simulink model "fi_afc"  (R2026a)
settings: Solver=ode15s  StopTime=simTime  FixedStep=5e-05  RelTol=1e-06  AbsTol=1e-06
undefined symbols (not defined in the file or in its folder): AF_sensor_tol, fault_time, fuel_inj_tol, MAF_sensor_tol, measureTime, simTime, spec_num
Description:
  | Modeling Engine Timing Using Triggered Subsystems
  | 
  | This example presents a model of a four-cylinder spark ignition engine
  | and demonstrates Simulink(R) capabilities to model an internal combustion
  | engine from the throttle to the crankshaft output. We used well-defined
  | physical principles supplemented, where appropriate, with empirical
  | relationships that describe the systems dynamic behavior without
  | introducing unnecessary complexity.
settings Model: ExtModeTrigMode=oneshot  ExtModeArmWhenConnect=off  ExtModeAutoUpdateStatusClock=off  Creator=The MathWorks Inc.  LastModifiedBy=harry_31916
settings SolverCC: ConsecutiveZCsStepRelTol=2.8421709430404e-13
settings DataIOCC: ExternalInput=[t__,u__]  InitialState=[]  LoadExternalInput=on  SaveFormat=StructureWithTime  SignalLoggingSaveFormat=ModelDataLogs  StateSaveName=x  SignalLoggingName=sldemo_engine_output
settings OptimizationCC: BooleanDataType=off  InitFltsAndDblsToZero=on  BufferReusableBoundary=off
settings DebuggingCC: SignalInfNanChecking=warning  SaveWithParameterizedLinksMsg=none  UnderspecifiedInitializationDetection=Classic  SignalResolutionControl=TryResolveAllWithWarning  InheritedTsInSrcMsg=none  MultiTaskDSMMsg=warning  MultiTaskCondExecSysMsg=none  SigSpecEnsureSampleTimeMsg=none  IntegerOverflowMsg=none  ParameterPrecisionLossMsg=none  UniqueDataStoreMsg=warning  IntegerSaturationMsg=none
settings HardwareCC: ProdHWDeviceType=32-bit Generic
settings GRTTargetCC: TargetFcnLib=ansi_tfl_tmw.mat  CombineOutputUpdateFcns=off  GRTInterface=on
settings ConfigComp: CovMetricSettings=d

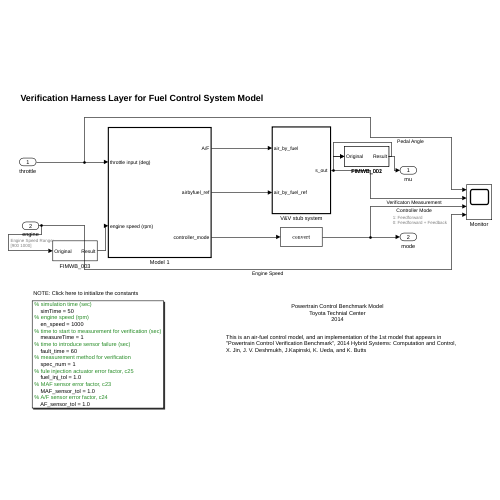
[thumbnail: Simulink's stored preview of the top-level diagram]
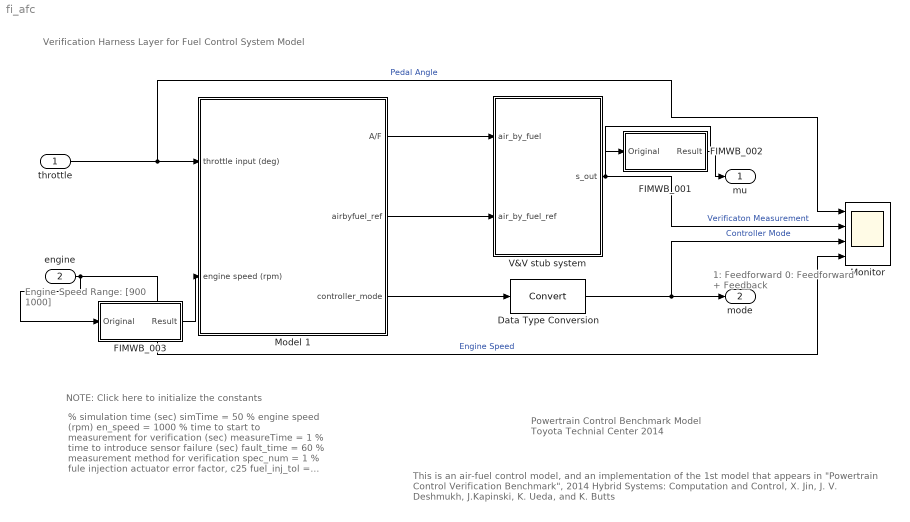
== system fi_afc ==
  note: 1: Feedforward
      | 0: Feedforward + Feedback
  note: NOTE: Click here to initialize the constants
  note: This is an air-fuel control model, and an implementation of the 1st model that appears in
      | "Powertrain Control Verification Benchmark", 2014 Hybrid Systems: Computation and Control,
      | X. Jin, J. V. Deshmukh, J.Kapinski, K. Ueda, and K. Butts
  note: % simulation time (sec)
      |     simTime = 50
      | % engine speed (rpm)
      |     en_speed = 1000
      | % time to start to measurement for verification (sec)
      |     measureTime = 1
      | % time to introduce sensor failure (sec)
      |     fault_time = 60
      | % measurement method for verification
      |     spec_num = 1
      | % fule injection actuator error factor, c25
      |     fuel_inj_tol = 1.0
      | % MAF sensor error factor, c23
      |     MAF_sensor_tol = 1.0
      | % A/F sensor error factor, c24
      |     AF_sensor_tol = 1.0
  note: Engine Speed Range:
      | [900 1000]
  note: Powertrain Control Benchmark Model
      | Toyota Technial Center
      | 2014
  note: Verification Harness Layer for Fuel Control System Model
  throttle : Inport  Interpolate=off
  engine : Inport  Port=2  Interpolate=off
  Data Type Conversion : DataTypeConversion  SaturateOnIntegerOverflow=off  RndMeth=Floor
  FIMWB_001 : Subsystem  Tag=fimwb.fault.1
  FIMWB_002 : Subsystem  Tag=fimwb.fault.2
  FIMWB_003 : Subsystem  Tag=fimwb.fault.3
  Model 1 : Subsystem  Priority=1  TreatAsAtomicUnit=on
  "Monitor " : Scope  NumInputPorts=4
      settings: TimeSpan=50  ActiveDisplayYMinimum=0  ActiveDisplayYMaximum=55
  V&V stub system : Subsystem  TreatAsAtomicUnit=on
  mu : Outport  VectorParamsAs1DForOutWhenUnconnected=off
  mode : Outport  Port=2  VectorParamsAs1DForOutWhenUnconnected=off
  wires:
  V&V stub system/1("s_out ") -> "Monitor "/2, FIMWB_001/1(Original)  "Verificaton Measurement"
  Model 1/1(A/F) -> V&V stub system/1("air_by_fuel ")
  engine/1 -> "Monitor "/4, FIMWB_003/1(Original)  "Engine Speed"
  throttle/1 -> "Monitor "/1, Model 1/1(throttle input (deg))  "Pedal Angle"
  Model 1/3(controller_mode) -> Data Type Conversion/1
  Data Type Conversion/1 -> "Monitor "/3, mode/1  "Controller Mode"
  Model 1/2(airbyfuel_ref) -> V&V stub system/2(air_by_fuel_ref)
  FIMWB_001/1(Result) -> FIMWB_002/1(Original)
  FIMWB_002/1(Result) -> mu/1
  FIMWB_003/1(Result) -> Model 1/2(engine speed (rpm))

== system fi_afc/FIMWB_001 ==
  Original : Inport
  Bias : Bias  Bias=-0.125  SaturateOnIntegerOverflow=off
  OutputType : DataTypeConversion  OutDataTypeStr=double  RndMeth=Round
  Result : Outport
  wires:
  Original/1 -> Bias/1
  Bias/1 -> OutputType/1
  OutputType/1 -> Result/1

== system fi_afc/FIMWB_002 ==
  Original : Inport
  Gain : Gain  Gain=1.5  OutDataTypeStr=Inherit: Same as input
  OutputType : DataTypeConversion  OutDataTypeStr=double  RndMeth=Round
  Result : Outport
  wires:
  Original/1 -> Gain/1
  Gain/1 -> OutputType/1
  OutputType/1 -> Result/1

== system fi_afc/FIMWB_003 ==
  Original : Inport
  Bias : Bias  Bias=0.015625  SaturateOnIntegerOverflow=off
  OutputType : DataTypeConversion  OutDataTypeStr=double  RndMeth=Round
  Result : Outport
  wires:
  Original/1 -> Bias/1
  Bias/1 -> OutputType/1
  OutputType/1 -> Result/1

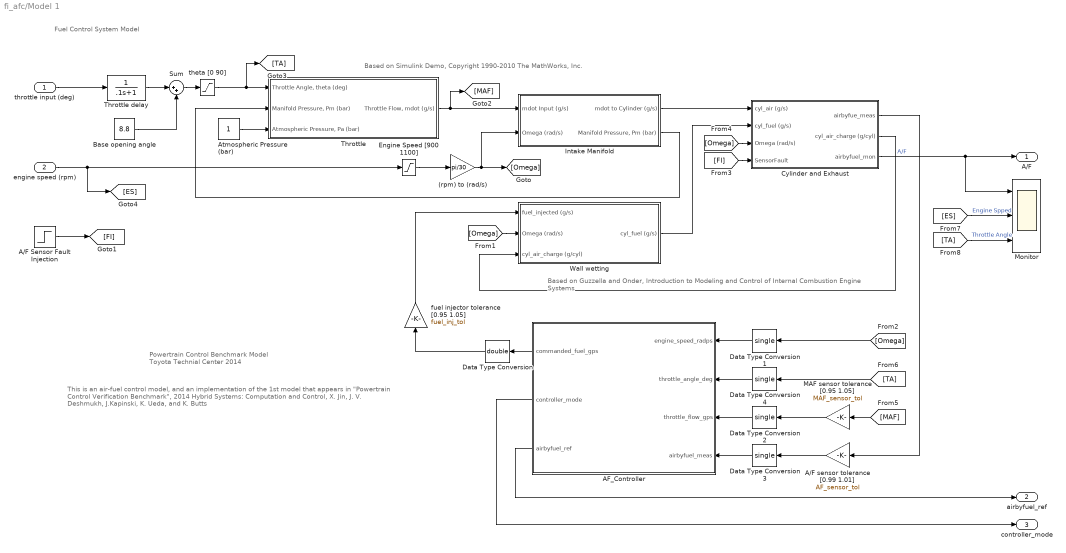
== system fi_afc/Model 1 ==
  note: Based on Simulink Demo, Copyright 1990-2010 The MathWorks, Inc.
  note: Based on Guzzella and Onder, Introduction to Modeling and Control of Internal Combustion Engine Systems
  note: Fuel Control System Model
  note: This is an air-fuel control model, and an implementation of the 1st model that appears in
      | "Powertrain Control Verification Benchmark", 2014 Hybrid Systems: Computation and Control,
      | X. Jin, J. V. Deshmukh, J.Kapinski, K. Ueda, and K. Butts
  note: Powertrain Control Benchmark Model
      | Toyota Technial Center
      | 2014
  throttle input (deg) : Inport  Description=[0, 81.2]
      settings: AttributesFormatString=%<Description>
  engine speed (rpm) : Inport  Description=[900,1100]  Port=2
      settings: AttributesFormatString=%<Description>
  (rpm) to (rad/s) : Gain  Gain=pi/30
  A/F Sensor Fault Injection : Step  Time=fault_time  SampleTime=0
      settings: AttributesFormatString=1: Failure\n0: Normal
  A/F sensor tolerance [0.99 1.01] : Gain  Gain=AF_sensor_tol
  AF_Controller : Subsystem  TreatAsAtomicUnit=on
  Atmospheric Pressure (bar) : Constant
  Base opening angle : Constant  Value=8.8
  Cylinder and Exhaust : Subsystem
  Data Type Conversion : DataTypeConversion  OutDataTypeStr=double  SaturateOnIntegerOverflow=off  RndMeth=Floor
  Data Type Conversion{1..4} (4 alike) : DataTypeConversion  OutDataTypeStr=single  SaturateOnIntegerOverflow=off  RndMeth=Floor
  Engine Speed [900 1100] : Saturate  UpperLimit=1100  LowerLimit=900
  Intake Manifold : Subsystem
  MAF sensor tolerance [0.95 1.05] : Gain  Gain=MAF_sensor_tol
  Monitor : Scope  NumInputPorts=3
      settings: TimeSpan=85  ActiveDisplayYMinimum=11.75  ActiveDisplayYMaximum=14.75
  Sum : Sum  Inputs=|++
  Throttle : Subsystem
  Throttle delay : TransferFcn  Denominator=[.1 1]
  Wall wetting : Subsystem
  fuel injector tolerance [0.95 1.05] : Gain  Gain=fuel_inj_tol
  theta [0 90] : Saturate  UpperLimit=90  LowerLimit=0
  A/F : Outport  VectorParamsAs1DForOutWhenUnconnected=off
  airbyfuel_ref : Outport  Port=2  VectorParamsAs1DForOutWhenUnconnected=off
  controller_mode : Outport  Port=3  VectorParamsAs1DForOutWhenUnconnected=off
  wires:
  (rpm) to (rad/s)/1 -> [Omega], Intake Manifold/2(Omega (rad/s))
  Data Type Conversion/1 -> fuel injector tolerance [0.95 1.05]/1
  theta [0 90]/1 -> Throttle/1("Throttle Angle, theta (deg)"), [TA]
  Engine Speed [900 1100]/1 -> (rpm) to (rad/s)/1
  Cylinder and Exhaust/3("airbyfuel_mon ") -> A/F/1, Monitor/1  "A/F"
  Data Type Conversion2/1 -> AF_Controller/3(throttle_flow_gps)
  Data Type Conversion3/1 -> AF_Controller/4(airbyfuel_meas)
  A/F sensor tolerance [0.99 1.01]/1 -> Data Type Conversion3/1
  [MAF] -> MAF sensor tolerance [0.95 1.05]/1
  Cylinder and Exhaust/1(airbyfue_meas) -> A/F sensor tolerance [0.99 1.01]/1
  Throttle/1("Throttle Flow, mdot (g/s)") -> [MAF], Intake Manifold/1(mdot Input (g/s))
  Intake Manifold/2("Manifold Pressure, Pm (bar)") -> Throttle/2("Manifold Pressure, Pm (bar)")
  Atmospheric Pressure (bar)/1 -> Throttle/3("Atmospheric Pressure, Pa (bar) ")
  Wall wetting/1(cyl_fuel (g/s)) -> Cylinder and Exhaust/2(cyl_fuel (g/s))
  Intake Manifold/1(mdot to Cylinder (g/s)) -> Cylinder and Exhaust/1(cyl_air (g/s))
  [Omega] -> Cylinder and Exhaust/3(Omega (rad/s))
  [Omega] -> Wall wetting/2(Omega (rad/s))
  Cylinder and Exhaust/2(cyl_air_charge (g/cyl)) -> Wall wetting/3(cyl_air_charge (g/cyl))
  [Omega] -> Data Type Conversion1/1
  fuel injector tolerance [0.95 1.05]/1 -> Wall wetting/1(fuel_injected (g/s))
  MAF sensor tolerance [0.95 1.05]/1 -> Data Type Conversion2/1
  AF_Controller/1(commanded_fuel_gps) -> Data Type Conversion/1
  Data Type Conversion1/1 -> AF_Controller/1(engine_speed_radps)
  A/F Sensor Fault Injection/1 -> [FI]
  [FI] -> Cylinder and Exhaust/4(SensorFault)
  [TA] -> Data Type Conversion4/1
  Data Type Conversion4/1 -> AF_Controller/2(throttle_angle_deg)
  throttle input (deg)/1 -> Throttle delay/1
  engine speed (rpm)/1 -> [ES], Engine Speed [900 1100]/1
  [TA] -> Monitor/3  "Throttle Angle"
  Throttle delay/1 -> Sum/1
  Base opening angle/1 -> Sum/2
  Sum/1 -> theta [0 90]/1
  AF_Controller/2(controller_mode) -> controller_mode/1
  AF_Controller/3(airbyfuel_ref) -> airbyfuel_ref/1
  [ES] -> Monitor/2  "Engine Spped"

== system fi_afc/V&V stub system ==
  "air_by_fuel " : Inport  OutDataTypeStr=double
  air_by_fuel_ref : Inport  Port=2
  Calcuate Error : Subsystem  Priority=20  TreatAsAtomicUnit=on
  Constant : Constant  Value=0.5
  Data Type Conversion : DataTypeConversion  OutDataTypeStr=double  SaturateOnIntegerOverflow=off  RndMeth=Floor
  MeasureOn : Step  Time=measureTime  SampleTime=0
  Relational Operator : RelationalOperator  Operator=>  OutDataTypeStr=boolean  InputSameDT=off
  spec_num : Constant  Value=spec_num  OutDataTypeStr=uint8
  "s_out " : Outport  VectorParamsAs1DForOutWhenUnconnected=off
  wires:
  Calcuate Error/1("s_out ") -> "s_out "/1
  MeasureOn/1 -> Relational Operator/1
  Constant/1 -> Relational Operator/2
  Relational Operator/1 -> Calcuate Error/Enable
  spec_num/1 -> Calcuate Error/2(spec_num)
  "air_by_fuel "/1 -> Calcuate Error/1("air_by_fuel ")
  air_by_fuel_ref/1 -> Data Type Conversion/1
  Data Type Conversion/1 -> Calcuate Error/3(air_by_fuel_ref)

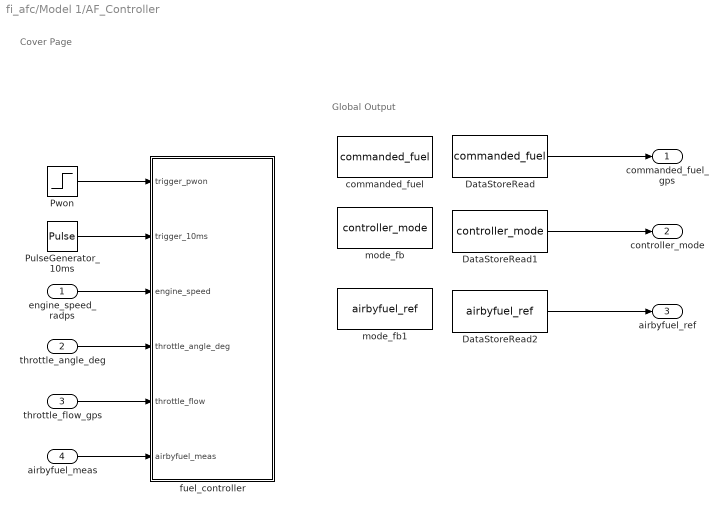
== system fi_afc/Model 1/AF_Controller ==
  note: Global Output
  note: Cover Page
  engine_speed_radps : Inport
  throttle_angle_deg : Inport  Port=2
  throttle_flow_gps : Inport  Port=3
  airbyfuel_meas : Inport  Port=4
  DataStoreRead : DataStoreRead  Priority=2  DataStoreName=commanded_fuel  IndexOptions=Index vector (dialog)  Indices=1  OutputSizes=1
  DataStoreRead1 : DataStoreRead  Priority=2  DataStoreName=controller_mode  IndexOptions=Index vector (dialog)  Indices=1  OutputSizes=1
  DataStoreRead2 : DataStoreRead  Priority=2  DataStoreName=airbyfuel_ref  IndexOptions=Index vector (dialog)  Indices=1  OutputSizes=1
  PulseGenerator_10ms : DiscretePulseGenerator  PulseType=Time based  Period=0.01  PulseWidth=50  PhaseDelay=0.01
  Pwon : Step  Time=0.001  SampleTime=0
  commanded_fuel : DataStoreMemory  DataStoreName=commanded_fuel  InitialValue=0.1726  ShowAdditionalParam=off  OutDataTypeStr=single
      settings: AttributesFormatString=commanded_fuel
  fuel_controller : Subsystem  Priority=1  TreatAsAtomicUnit=on
      settings: AttributesFormatString=Priority = %<Priority>
  mode_fb : DataStoreMemory  DataStoreName=controller_mode  ShowAdditionalParam=off  OutDataTypeStr=boolean
      settings: AttributesFormatString=controller_mode
  mode_fb1 : DataStoreMemory  DataStoreName=airbyfuel_ref  ShowAdditionalParam=off  OutDataTypeStr=single
  commanded_fuel_gps : Outport  VectorParamsAs1DForOutWhenUnconnected=off
  controller_mode : Outport  Port=2  VectorParamsAs1DForOutWhenUnconnected=off
  airbyfuel_ref : Outport  Port=3  VectorParamsAs1DForOutWhenUnconnected=off
  wires:
  DataStoreRead/1 -> commanded_fuel_gps/1
  airbyfuel_meas/1 -> fuel_controller/6(airbyfuel_meas)
  throttle_flow_gps/1 -> fuel_controller/5(throttle_flow)
  engine_speed_radps/1 -> fuel_controller/3(engine_speed)
  Pwon/1 -> fuel_controller/1(trigger_pwon)
  throttle_angle_deg/1 -> fuel_controller/4(throttle_angle_deg)
  PulseGenerator_10ms/1 -> fuel_controller/2(trigger_10ms)
  DataStoreRead1/1 -> controller_mode/1
  DataStoreRead2/1 -> airbyfuel_ref/1

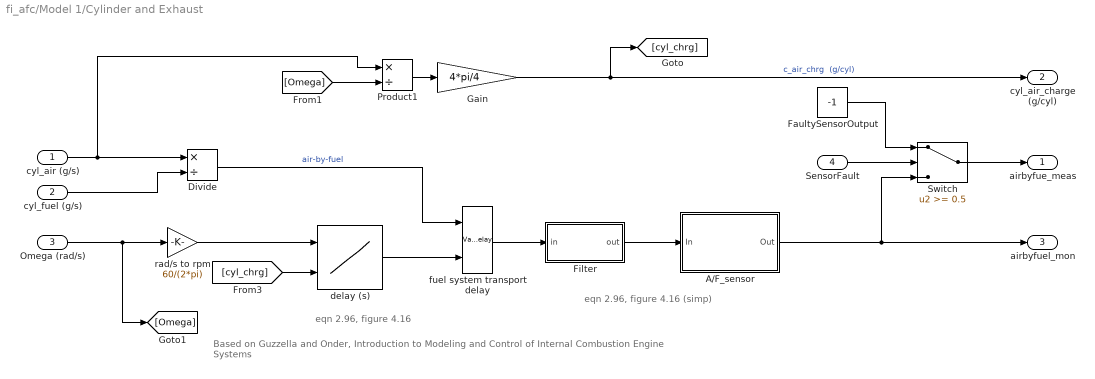
== system fi_afc/Model 1/Cylinder and Exhaust ==
  note: Based on Guzzella and Onder, Introduction to Modeling and Control of Internal Combustion Engine Systems
  note: eqn 2.96, figure 4.16
  note: eqn 2.96, figure 4.16 (simp)
  cyl_air (g/s) : Inport
  cyl_fuel (g/s) : Inport  Port=2
  Omega (rad/s) : Inport  Port=3
  SensorFault : Inport  Port=4
  A/F_sensor : Subsystem
  Divide : Product  Inputs=*/
  FaultySensorOutput : Constant  Value=-1
  Filter : Subsystem
  Gain : Gain  Gain=4*pi/4
  Product1 : Product  Inputs=*/  RndMeth=Zero
  Switch : Switch  Threshold=0.5  SaturateOnIntegerOverflow=off  InputSameDT=off
  delay (s) : Lookup_n-D  BreakpointsForDimension1=[800,1000,1500,2000,3000]  BreakpointsForDimension2=[0.05,0.15,0.2,0.25]  Table=reshape([0.8,0.6,0.4,0.3,0.2,0.4,0.3,0.2,0.2,0.2,0.3,0.25,0.2,0.2,0.2,0.25,0.2,0.2,0.2,0.2],5,4)  UseLastTableValue=on  RndMeth=Simplest
      settings: InputPortMap=u0,u1
  fuel system transport delay : VariableTransportDelay  VariableDelayType=Variable transport delay  MaximumDelay=10  InitialOutput=14.7  MaximumPoints=20480
  rad/s to rpm : Gain  Gain=60/(2*pi)
  airbyfue_meas : Outport  VectorParamsAs1DForOutWhenUnconnected=off
  cyl_air_charge (g/cyl) : Outport  Port=2  VectorParamsAs1DForOutWhenUnconnected=off
  "airbyfuel_mon " : Outport  Port=3  VectorParamsAs1DForOutWhenUnconnected=off
  wires:
  cyl_air (g/s)/1 -> Divide/1, Product1/1
  [Omega] -> Product1/2
  Product1/1 -> Gain/1
  Gain/1 -> [cyl_chrg], cyl_air_charge (g/cyl)/1  "c_air_chrg  (g/cyl)"
  [cyl_chrg] -> delay (s)/2
  cyl_fuel (g/s)/1 -> Divide/2
  Omega (rad/s)/1 -> [Omega], rad/s to rpm/1
  rad/s to rpm/1 -> delay (s)/1
  delay (s)/1 -> fuel system transport delay/2
  fuel system transport delay/1 -> Filter/1(in)
  Switch/1 -> airbyfue_meas/1
  Divide/1 -> fuel system transport delay/1  "air-by-fuel"
  Filter/1(out) -> A/F_sensor/1(In)
  FaultySensorOutput/1 -> Switch/1
  SensorFault/1 -> Switch/2
  A/F_sensor/1(Out) -> Switch/3, "airbyfuel_mon "/1

== system fi_afc/Model 1/Intake Manifold ==
  note: Intake Manifold Vacuum
  note: Based on Simulink Demo, Copyright 1990-2010 The MathWorks, Inc.
  mdot Input (g/s) : Inport
  Omega (rad/s) : Inport  Port=2
  Gain2 : Gain  Gain=0.9  ParamDataTypeStr=single  OutDataTypeStr=Inherit: Inherit via back propagation  RndMeth=Simplest  SaturateOnIntegerOverflow=on
      settings: AttributesFormatString=pumping tolerance [0.9 1.1]
  Mux : Mux  Inputs=2
  Pumping : Fcn  Expr=-0.366 + 0.08979*u[1]*u[2] - 0.0337*u[2]*u[1]*u[1] + 0.0001*u[1]*u[2]*u[2]
  RT/Vm : Gain  Gain=0.41328  SaturateOnIntegerOverflow=on  OutDataTypeStr=Inherit: Same as input  ParamDataTypeStr=Inherit: Same as input
  Sum : Sum  Inputs=|+-  InputSameDT=on  SaturateOnIntegerOverflow=on  OutDataTypeStr=Inherit: Same as first input
  p0 = 0.543 (bar) : Integrator  InitialCondition=0.982
  mdot to Cylinder (g/s) : Outport  InitialOutput=0  VectorParamsAs1DForOutWhenUnconnected=off
  "Manifold Pressure, Pm (bar)" : Outport  Port=2  InitialOutput=0  VectorParamsAs1DForOutWhenUnconnected=off
  wires:
  mdot Input (g/s)/1 -> Sum/1
  RT/Vm/1 -> p0 = 0.543 (bar)/1
  Omega (rad/s)/1 -> Mux/2
  Mux/1 -> Pumping/1
  p0 = 0.543 (bar)/1 -> Mux/1, "Manifold Pressure, Pm (bar)"/1
  Sum/1 -> RT/Vm/1
  Pumping/1 -> Gain2/1
  Gain2/1 -> Sum/2, mdot to Cylinder (g/s)/1

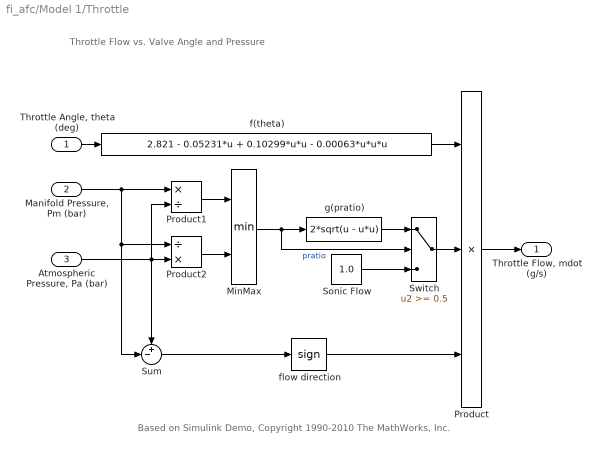
== system fi_afc/Model 1/Throttle ==
  note: Throttle Flow vs. Valve Angle and Pressure
  note: Based on Simulink Demo, Copyright 1990-2010 The MathWorks, Inc.
  "Throttle Angle, theta (deg)" : Inport
  "Manifold Pressure, Pm (bar)" : Inport  Port=2
  "Atmospheric Pressure, Pa (bar) " : Inport  Port=3
  MinMax : MinMax  Inputs=2  InputSameDT=on  SaturateOnIntegerOverflow=on
  Product : Product  Inputs=3  InputSameDT=on  RndMeth=Zero  SaturateOnIntegerOverflow=on  OutDataTypeStr=Inherit: Same as first input
  Product1 : Product  Inputs=*/  InputSameDT=on  RndMeth=Zero  SaturateOnIntegerOverflow=on  OutDataTypeStr=Inherit: Same as first input
  Product2 : Product  Inputs=/*  InputSameDT=on  RndMeth=Zero  SaturateOnIntegerOverflow=on  OutDataTypeStr=Inherit: Same as first input
  "Sonic Flow " : Constant  Value=1.0
  Sum : Sum  Inputs=+-|  InputSameDT=on  SaturateOnIntegerOverflow=on  OutDataTypeStr=Inherit: Same as first input
  Switch : Switch  Threshold=0.5
  f(theta) : Fcn  Expr=2.821 - 0.05231*u + 0.10299*u*u - 0.00063*u*u*u
  flow direction : Signum
  g(pratio) : Fcn  Expr=2*sqrt(u - u*u)
  "Throttle Flow, mdot (g/s)" : Outport  InitialOutput=0  VectorParamsAs1DForOutWhenUnconnected=off
  wires:
  "Manifold Pressure, Pm (bar)"/1 -> Sum/2, Product2/1, Product1/1
  Product2/1 -> MinMax/2
  Product1/1 -> MinMax/1
  "Atmospheric Pressure, Pa (bar) "/1 -> Sum/1, Product2/2, Product1/2
  g(pratio)/1 -> Switch/1
  "Sonic Flow "/1 -> Switch/3
  Switch/1 -> Product/2
  flow direction/1 -> Product/3
  Sum/1 -> flow direction/1
  MinMax/1 -> g(pratio)/1, Switch/2  "pratio"
  "Throttle Angle, theta (deg)"/1 -> f(theta)/1
  Product/1 -> "Throttle Flow, mdot (g/s)"/1
  f(theta)/1 -> Product/1

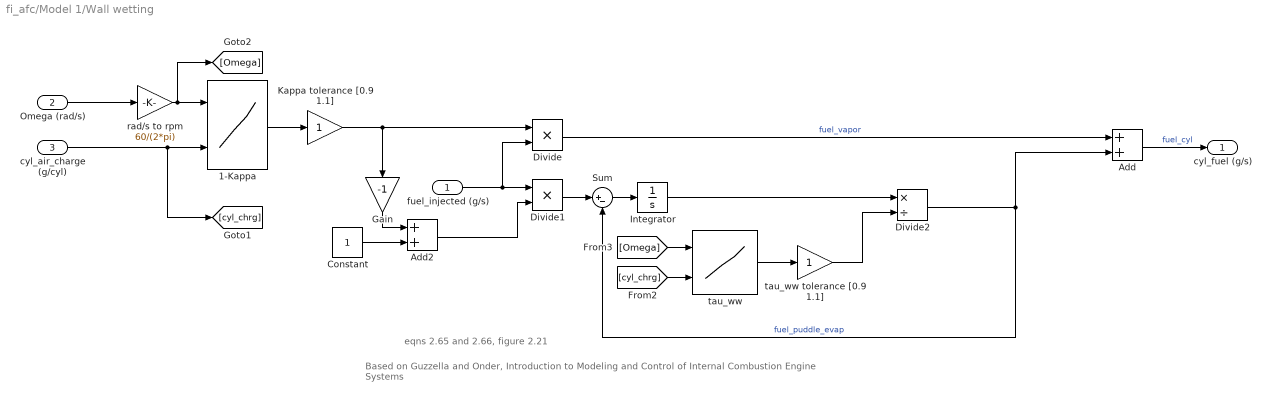
== system fi_afc/Model 1/Wall wetting ==
  note: Based on Guzzella and Onder, Introduction to Modeling and Control of Internal Combustion Engine Systems
  note: eqns 2.65 and 2.66, figure 2.21
  fuel_injected (g/s) : Inport
  Omega (rad/s) : Inport  Port=2
  cyl_air_charge (g/cyl) : Inport  Port=3
  1-Kappa : Lookup_n-D  BreakpointsForDimension1=[1000,1500,2000,2500,3000]  BreakpointsForDimension2=[.1,.2,.3,.4]  Table=reshape([0.8,.7,.7,.8,.9,.7,.66,.65,.73,.85,.66,.66,.63,.66,.8,.6,.6,.6,.6,.7],5,4)  UseLastTableValue=on  RndMeth=Simplest
      settings: InputPortMap=u0,u1
  Add : Sum
  Add2 : Sum
  Constant : Constant
  Divide : Product  Inputs=**
  Divide1 : Product  Inputs=**
  Divide2 : Product  Inputs=*/
  Gain : Gain  Gain=-1
  Integrator : Integrator  InitialCondition=.0112
  Kappa tolerance [0.9 1.1] : Gain
  Sum : Sum  Inputs=|+-
  rad/s to rpm : Gain  Gain=60/(2*pi)
  tau_ww : Lookup_n-D  BreakpointsForDimension1=[1000,1500,2000,2500,3000]  BreakpointsForDimension2=[0.1,0.2,0.3,0.4]  Table=reshape([.4,.3,.35,.3,.2,.22,.22,.4,.35,.5,.20,.22,.5,.4,.35,.35,.3,.45,.5,.4],5,4)  UseLastTableValue=on  RndMeth=Simplest
      settings: InputPortMap=u0,u1
  tau_ww tolerance [0.9 1.1] : Gain
  cyl_fuel (g/s) : Outport  VectorParamsAs1DForOutWhenUnconnected=off
  wires:
  1-Kappa/1 -> Kappa tolerance [0.9 1.1]/1
  fuel_injected (g/s)/1 -> Divide/2, Divide1/1
  Divide/1 -> Add/1  "fuel_vapor"
  Add/1 -> cyl_fuel (g/s)/1  "fuel_cyl"
  Integrator/1 -> Divide2/1
  Divide1/1 -> Sum/1
  Sum/1 -> Integrator/1
  Divide2/1 -> Add/2, Sum/2  "fuel_puddle_evap"
  Add2/1 -> Divide1/2
  cyl_air_charge (g/cyl)/1 -> 1-Kappa/2, [cyl_chrg]
  [cyl_chrg] -> tau_ww/2
  tau_ww/1 -> tau_ww tolerance [0.9 1.1]/1
  Gain/1 -> Add2/1
  Constant/1 -> Add2/2
  rad/s to rpm/1 -> [Omega], 1-Kappa/1
  Omega (rad/s)/1 -> rad/s to rpm/1
  Kappa tolerance [0.9 1.1]/1 -> Divide/1, Gain/1
  tau_ww tolerance [0.9 1.1]/1 -> Divide2/2
  [Omega] -> tau_ww/1

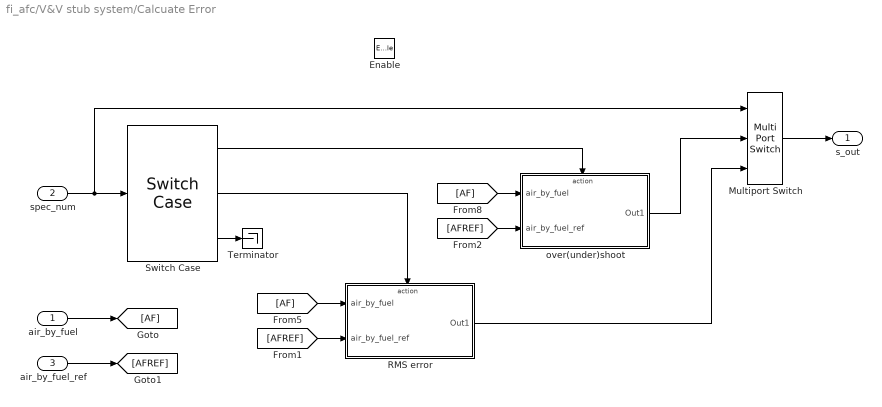
== system fi_afc/V&V stub system/Calcuate Error ==
  "air_by_fuel " : Inport
  spec_num : Inport  Port=2  OutDataTypeStr=uint8
  air_by_fuel_ref : Inport  Port=3
  Enable : EnablePort
  Multiport Switch : MultiPortSwitch  Inputs=2  SaturateOnIntegerOverflow=off  InputSameDT=off
  RMS error : Subsystem  TreatAsAtomicUnit=on
  Switch Case : SwitchCase  CaseConditions={1,2}
  Terminator : Terminator
  over(under)shoot : Subsystem  TreatAsAtomicUnit=on
  "s_out " : Outport  VectorParamsAs1DForOutWhenUnconnected=off
  wires:
  "air_by_fuel "/1 -> [AF]
  spec_num/1 -> Multiport Switch/1, Switch Case/1
  Switch Case/1 -> over(under)shoot/Action
  [AF] -> over(under)shoot/1("air_by_fuel ")
  Switch Case/2 -> RMS error/Action
  [AF] -> RMS error/1("air_by_fuel ")
  Multiport Switch/1 -> "s_out "/1
  over(under)shoot/1(Out1) -> Multiport Switch/2
  RMS error/1(Out1) -> Multiport Switch/3
  Switch Case/3 -> Terminator/1
  air_by_fuel_ref/1 -> [AFREF]
  [AFREF] -> over(under)shoot/2(air_by_fuel_ref)
  [AFREF] -> RMS error/2(air_by_fuel_ref)

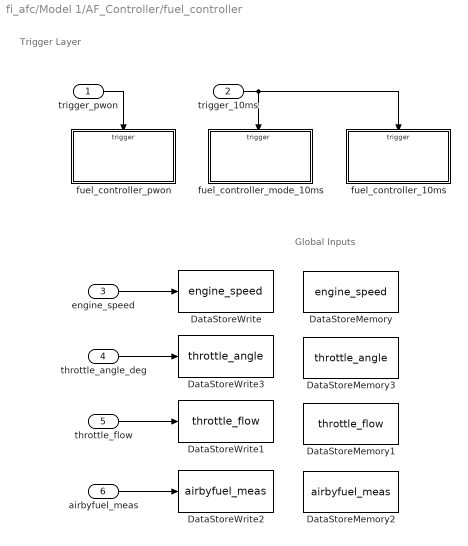
== system fi_afc/Model 1/AF_Controller/fuel_controller ==
  note: Global Inputs
  note: Trigger Layer
  trigger_pwon : Inport
  trigger_10ms : Inport  Port=2
  engine_speed : Inport  Port=3
  throttle_angle_deg : Inport  Port=4
  throttle_flow : Inport  Port=5
  airbyfuel_meas : Inport  Port=6
  DataStoreMemory : DataStoreMemory  DataStoreName=engine_speed  ShowAdditionalParam=off  OutDataTypeStr=single
      settings: AttributesFormatString=engine speed
  DataStoreMemory1 : DataStoreMemory  DataStoreName=throttle_flow  ShowAdditionalParam=off  OutDataTypeStr=single
      settings: AttributesFormatString=throttle flow
  DataStoreMemory2 : DataStoreMemory  DataStoreName=airbyfuel_meas  ShowAdditionalParam=off  OutDataTypeStr=single
      settings: AttributesFormatString=lambda_meas
  DataStoreMemory3 : DataStoreMemory  DataStoreName=throttle_angle  ShowAdditionalParam=off  OutDataTypeStr=single
      settings: AttributesFormatString=throttle flow
  DataStoreWrite : DataStoreWrite  Priority=1  DataStoreName=engine_speed  IndexOptions=Index vector (dialog)  Indices=1  OutputSizes=1
  DataStoreWrite1 : DataStoreWrite  Priority=1  DataStoreName=throttle_flow  IndexOptions=Index vector (dialog)  Indices=1  OutputSizes=1
  DataStoreWrite2 : DataStoreWrite  Priority=1  DataStoreName=airbyfuel_meas  IndexOptions=Index vector (dialog)  Indices=1  OutputSizes=1
  DataStoreWrite3 : DataStoreWrite  Priority=1  DataStoreName=throttle_angle  IndexOptions=Index vector (dialog)  Indices=1  OutputSizes=1
  fuel_controller_10ms : Subsystem  Priority=30  TreatAsAtomicUnit=on
      settings: AttributesFormatString=Priority = %<Priority>
  fuel_controller_mode_10ms : Subsystem  Priority=20  TreatAsAtomicUnit=on
      settings: AttributesFormatString=Priority = %<Priority>
  fuel_controller_pwon : Subsystem  Priority=10  TreatAsAtomicUnit=on
      settings: AttributesFormatString=Priority = %<Priority>
  wires:
  airbyfuel_meas/1 -> DataStoreWrite2/1
  throttle_flow/1 -> DataStoreWrite1/1
  engine_speed/1 -> DataStoreWrite/1
  trigger_10ms/1 -> fuel_controller_mode_10ms/Trigger, fuel_controller_10ms/Trigger
  trigger_pwon/1 -> fuel_controller_pwon/Trigger
  throttle_angle_deg/1 -> DataStoreWrite3/1

== system fi_afc/Model 1/Cylinder and Exhaust/A//F_sensor ==
  In : Inport
  A/F_sensor : Gain  OutDataTypeStr=double
  Filter : Subsystem
  Out : Outport  VectorParamsAs1DForOutWhenUnconnected=off
  wires:
  A/F_sensor/1 -> Out/1
  In/1 -> Filter/1(In)
  Filter/1(Out) -> A/F_sensor/1

== system fi_afc/Model 1/Cylinder and Exhaust/Filter ==
  in : Inport
  Gain1 : Gain  Gain=10
  Integrator : Integrator  InitialCondition=14.7
  Sum : Sum  Inputs=|+-
  out : Outport  VectorParamsAs1DForOutWhenUnconnected=off
  wires:
  Integrator/1 -> out/1, Sum/2
  in/1 -> Sum/1
  Gain1/1 -> Integrator/1
  Sum/1 -> Gain1/1

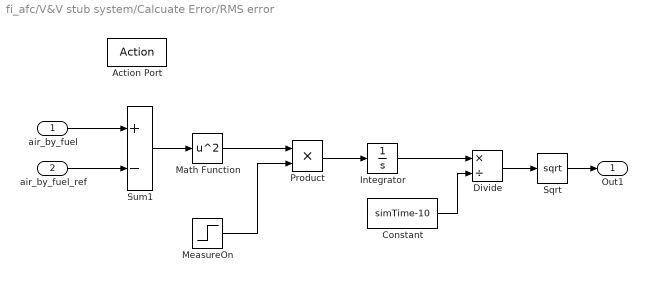
== system fi_afc/V&V stub system/Calcuate Error/RMS error ==
  "air_by_fuel " : Inport
  air_by_fuel_ref : Inport  Port=2
  Action Port : ActionPort  ActionPortLabel=case [ 2 ]:
  Constant : Constant  Value=simTime-10
  Divide : Product  Inputs=*/
  Integrator : Integrator
  Math Function : Math  Operator=square  SignedPower=on
  MeasureOn : Step  Time=10  SampleTime=0
  Product : Product
  Sqrt : Sqrt
  Sum1 : Sum  Inputs=+-  OutDataTypeStr=Inherit: Inherit via back propagation  InputSameDT=on  RndMeth=Simplest
  Out1 : Outport  VectorParamsAs1DForOutWhenUnconnected=off
  wires:
  Sum1/1 -> Math Function/1
  Math Function/1 -> Product/1
  "air_by_fuel "/1 -> Sum1/1
  Divide/1 -> Sqrt/1
  Constant/1 -> Divide/2
  air_by_fuel_ref/1 -> Sum1/2
  MeasureOn/1 -> Product/2
  Product/1 -> Integrator/1
  Integrator/1 -> Divide/1
  Sqrt/1 -> Out1/1

== system fi_afc/V&V stub system/Calcuate Error/over(under)shoot ==
  "air_by_fuel " : Inport
  air_by_fuel_ref : Inport  Port=2
  Action Port : ActionPort  ActionPortLabel=case [ 1 ]:
  Constant : Constant
  Divide : Product  Inputs=*/
  Sum1 : Sum  Inputs=+-  OutDataTypeStr=Inherit: Inherit via back propagation  InputSameDT=on  RndMeth=Simplest
  Out1 : Outport  VectorParamsAs1DForOutWhenUnconnected=off
  wires:
  "air_by_fuel "/1 -> Divide/1
  Divide/1 -> Sum1/1
  Constant/1 -> Sum1/2
  Sum1/1 -> Out1/1
  air_by_fuel_ref/1 -> Divide/2

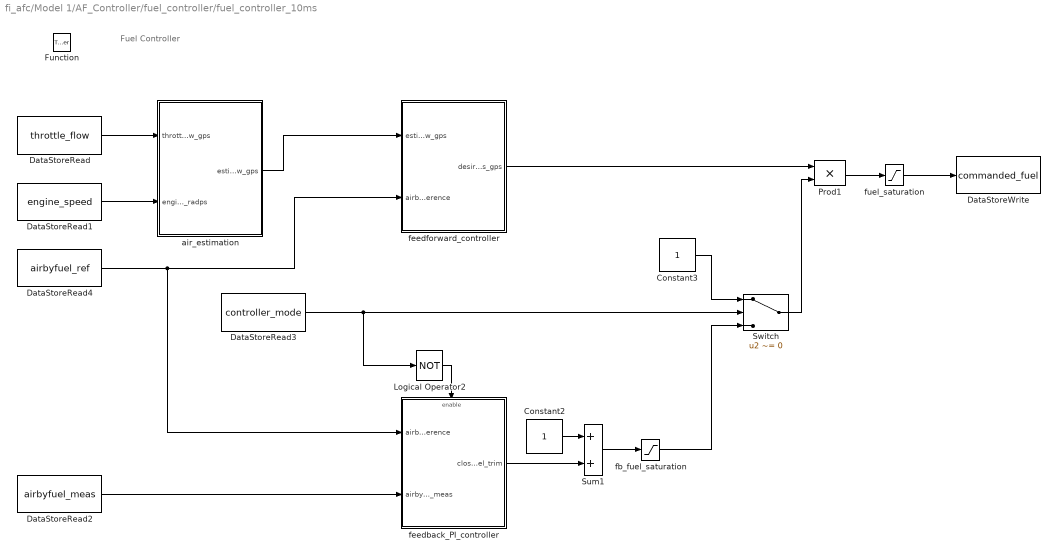
== system fi_afc/Model 1/AF_Controller/fuel_controller/fuel_controller_10ms ==
  note: Fuel Controller
  Function : TriggerPort  VariantControl=(inherit)
  Constant2 : Constant  OutDataTypeStr=single
  Constant3 : Constant  OutDataTypeStr=single
  DataStoreRead : DataStoreRead  DataStoreName=throttle_flow  IndexOptions=Index vector (dialog)  Indices=1  OutputSizes=1
  DataStoreRead1 : DataStoreRead  DataStoreName=engine_speed  IndexOptions=Index vector (dialog)  Indices=1  OutputSizes=1
  DataStoreRead2 : DataStoreRead  DataStoreName=airbyfuel_meas  IndexOptions=Index vector (dialog)  Indices=1  OutputSizes=1
  DataStoreRead3 : DataStoreRead  DataStoreName=controller_mode  IndexOptions=Index vector (dialog)  Indices=1  OutputSizes=1
      settings: AttributesFormatString=1: Feedforward\n0: Feedforward + Feedback
  DataStoreRead4 : DataStoreRead  DataStoreName=airbyfuel_ref  IndexOptions=Index vector (dialog)  Indices=1  OutputSizes=1
  DataStoreWrite : DataStoreWrite  DataStoreName=commanded_fuel  IndexOptions=Index vector (dialog)  Indices=1  OutputSizes=1
  Logical Operator2 : Logic  Operator=NOT  AllPortsSameDT=off  OutDataTypeStr=boolean
  Prod1 : Product  OutDataTypeStr=Inherit: Inherit via back propagation  RndMeth=Simplest
  Sum1 : Sum  OutDataTypeStr=Inherit: Inherit via back propagation  InputSameDT=on  RndMeth=Simplest
  Switch : Switch  Criteria=u2 ~= 0  Threshold=0.5  SaturateOnIntegerOverflow=off  InputSameDT=off
  air_estimation : Subsystem  TreatAsAtomicUnit=on
  fb_fuel_saturation : Saturate  UpperLimit=inf  LowerLimit=0  RndMeth=Round
      settings: AttributesFormatString=y >= 0
  feedback_PI_controller : Subsystem  TreatAsAtomicUnit=on
  feedforward_controller : Subsystem  TreatAsAtomicUnit=on
  fuel_saturation : Saturate  UpperLimit=1.66  LowerLimit=0.13  RndMeth=Round
      settings: AttributesFormatString=0.13 <=\ncommanded_fuel\n<= 1.66
  wires:
  DataStoreRead4/1 -> feedback_PI_controller/1(airbyfuel_reference), feedforward_controller/2(airbyfuel_reference)
  Prod1/1 -> fuel_saturation/1
  feedforward_controller/1(desired_fuel_mass_gps) -> Prod1/1
  feedback_PI_controller/1(closed_loop_fuel_trim) -> Sum1/2
  Constant2/1 -> Sum1/1
  air_estimation/1(estimated_cyl_air_flow_gps) -> feedforward_controller/1(estimated_cyl_air_flow_gps)
  DataStoreRead1/1 -> air_estimation/2(engine_speed_radps)
  DataStoreRead/1 -> air_estimation/1(throttle_flow_gps)
  Sum1/1 -> fb_fuel_saturation/1
  Switch/1 -> Prod1/2
  fuel_saturation/1 -> DataStoreWrite/1
  DataStoreRead3/1 -> Logical Operator2/1, Switch/2
  Constant3/1 -> Switch/1
  fb_fuel_saturation/1 -> Switch/3
  Logical Operator2/1 -> feedback_PI_controller/Enable
  DataStoreRead2/1 -> feedback_PI_controller/2(airbyfuel_meas)

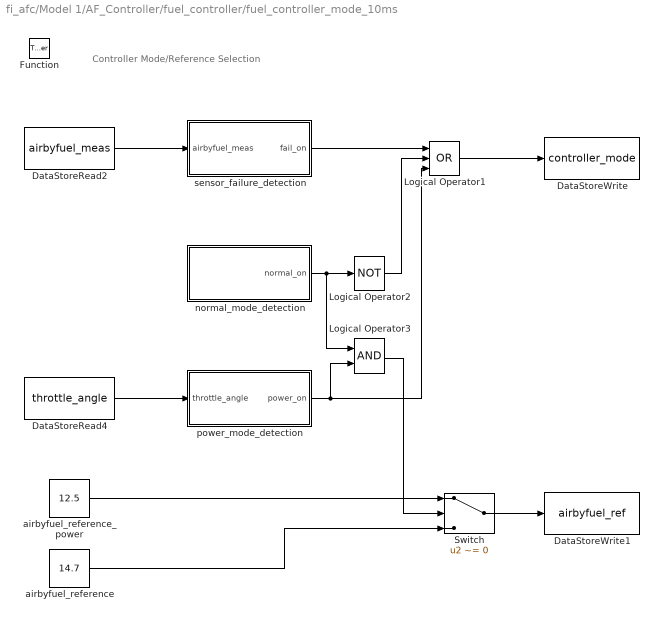
== system fi_afc/Model 1/AF_Controller/fuel_controller/fuel_controller_mode_10ms ==
  note: Controller Mode/Reference Selection
  Function : TriggerPort  VariantControl=(inherit)
  DataStoreRead2 : DataStoreRead  DataStoreName=airbyfuel_meas  IndexOptions=Index vector (dialog)  Indices=1  OutputSizes=1
  DataStoreRead4 : DataStoreRead  DataStoreName=throttle_angle  IndexOptions=Index vector (dialog)  Indices=1  OutputSizes=1
  DataStoreWrite : DataStoreWrite  DataStoreName=controller_mode  IndexOptions=Index vector (dialog)  Indices=1  OutputSizes=1
      settings: AttributesFormatString=1: Feedforward\n0: Feedforward + Feedback
  DataStoreWrite1 : DataStoreWrite  DataStoreName=airbyfuel_ref  IndexOptions=Index vector (dialog)  Indices=1  OutputSizes=1
  Logical Operator1 : Logic  Operator=OR  Inputs=3  AllPortsSameDT=off  OutDataTypeStr=boolean
  Logical Operator2 : Logic  Operator=NOT  AllPortsSameDT=off  OutDataTypeStr=boolean
  Logical Operator3 : Logic  AllPortsSameDT=off  OutDataTypeStr=boolean
  Switch : Switch  Criteria=u2 ~= 0  SaturateOnIntegerOverflow=off  InputSameDT=off
  airbyfuel_reference : Constant  Value=14.7  OutDataTypeStr=single  SampleTime=-1
  airbyfuel_reference_power : Constant  Value=12.5  OutDataTypeStr=single  SampleTime=-1
  normal_mode_detection : Subsystem  TreatAsAtomicUnit=on
      settings: AttributesFormatString=0: Feedforward\n1: Feedforward + Feedback
  power_mode_detection : Subsystem  TreatAsAtomicUnit=on
      settings: AttributesFormatString=1: Feedforward\n0: Feedforward + Feedback
  sensor_failure_detection : Subsystem  TreatAsAtomicUnit=on
      settings: AttributesFormatString=1: Feedforward\n0: Feedforward + Feedback
  wires:
  sensor_failure_detection/1(fail_on) -> Logical Operator1/1
  DataStoreRead4/1 -> power_mode_detection/1(throttle_angle)
  DataStoreRead2/1 -> sensor_failure_detection/1(airbyfuel_meas)
  Logical Operator1/1 -> DataStoreWrite/1
  normal_mode_detection/1(normal_on) -> Logical Operator3/1, Logical Operator2/1
  Switch/1 -> DataStoreWrite1/1
  power_mode_detection/1(power_on) -> Logical Operator3/2, Logical Operator1/3
  Logical Operator2/1 -> Logical Operator1/2
  airbyfuel_reference_power/1 -> Switch/1
  airbyfuel_reference/1 -> Switch/3
  Logical Operator3/1 -> Switch/2

== system fi_afc/Model 1/AF_Controller/fuel_controller/fuel_controller_pwon ==
  Function : TriggerPort  VariantControl=(inherit)
  Constant1 : Constant  OutDataTypeStr=single  SampleTime=-1
  Constant2 : Constant  Value=0.1726  OutDataTypeStr=single  SampleTime=-1
  Constant3 : Constant  Value=14.7  OutDataTypeStr=single  SampleTime=-1
  Data Type Conversion : DataTypeConversion  OutDataTypeStr=boolean  SaturateOnIntegerOverflow=off  RndMeth=Floor
  DataStoreWrite : DataStoreWrite  DataStoreName=commanded_fuel  IndexOptions=Index vector (dialog)  Indices=1  OutputSizes=1
  DataStoreWrite1 : DataStoreWrite  DataStoreName=controller_mode  IndexOptions=Index vector (dialog)  Indices=1  OutputSizes=1
  DataStoreWrite2 : DataStoreWrite  DataStoreName=airbyfuel_ref  IndexOptions=Index vector (dialog)  Indices=1  OutputSizes=1
  wires:
  Constant2/1 -> DataStoreWrite/1
  Constant1/1 -> Data Type Conversion/1
  Constant3/1 -> DataStoreWrite2/1
  Data Type Conversion/1 -> DataStoreWrite1/1

== system fi_afc/Model 1/Cylinder and Exhaust/A//F_sensor/Filter ==
  In : Inport
  Gain : Gain  Gain=50
  Integrator : Integrator  InitialCondition=14.7
  Sum : Sum  Inputs=|+-
  Out : Outport  VectorParamsAs1DForOutWhenUnconnected=off
  wires:
  Integrator/1 -> Out/1, Sum/2
  In/1 -> Sum/1
  Gain/1 -> Integrator/1
  Sum/1 -> Gain/1

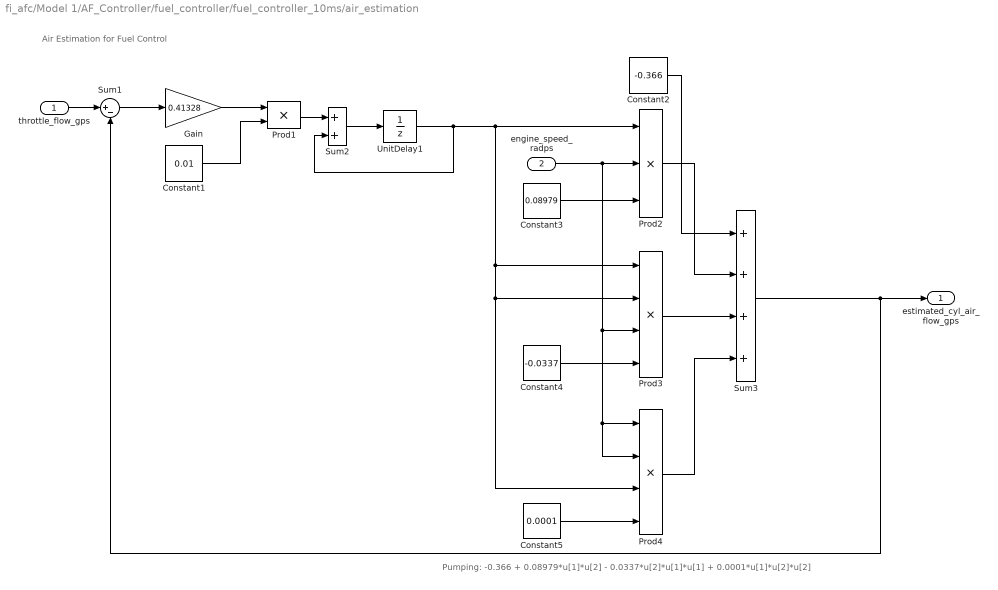
== system fi_afc/Model 1/AF_Controller/fuel_controller/fuel_controller_10ms/air_estimation ==
  note: Air Estimation for Fuel Control
  note: Pumping: -0.366 + 0.08979*u[1]*u[2] - 0.0337*u[2]*u[1]*u[1] + 0.0001*u[1]*u[2]*u[2]
  throttle_flow_gps : Inport
  engine_speed_radps : Inport  Port=2
  Constant1 : Constant  Value=0.01  OutDataTypeStr=single  SampleTime=-1
      settings: AttributesFormatString=Sample Time (s)
  Constant2 : Constant  Value=-0.366  OutDataTypeStr=single  SampleTime=-1
  Constant3 : Constant  Value=0.08979  OutDataTypeStr=single  SampleTime=-1
  Constant4 : Constant  Value=-0.0337  OutDataTypeStr=single  SampleTime=-1
  Constant5 : Constant  Value=0.0001  OutDataTypeStr=single  SampleTime=-1
  Gain : Gain  Gain=0.41328  ParamDataTypeStr=single  OutDataTypeStr=Inherit: Inherit via back propagation  RndMeth=Simplest  SaturateOnIntegerOverflow=on
      settings: AttributesFormatString=RT/Vm
  Prod1 : Product  OutDataTypeStr=Inherit: Inherit via back propagation  RndMeth=Simplest
  Prod2 : Product  Inputs=3  OutDataTypeStr=Inherit: Inherit via back propagation  RndMeth=Simplest
  Prod3 : Product  Inputs=4  OutDataTypeStr=Inherit: Inherit via back propagation  RndMeth=Simplest
  Prod4 : Product  Inputs=4  OutDataTypeStr=Inherit: Inherit via back propagation  RndMeth=Simplest
  Sum1 : Sum  Inputs=|+-  OutDataTypeStr=Inherit: Inherit via back propagation  InputSameDT=on  RndMeth=Simplest
  Sum2 : Sum  OutDataTypeStr=Inherit: Inherit via back propagation  InputSameDT=on  RndMeth=Simplest
  Sum3 : Sum  Inputs=++++  OutDataTypeStr=Inherit: Inherit via back propagation  InputSameDT=on  RndMeth=Simplest
  UnitDelay1 : UnitDelay  InitialCondition=0.982  SampleTime=-1
      settings: AttributesFormatString=p0 = %<InitialCondition> (bar)
  estimated_cyl_air_flow_gps : Outport  VectorParamsAs1DForOutWhenUnconnected=off
  wires:
  Sum3/1 -> Sum1/2, estimated_cyl_air_flow_gps/1
  Constant5/1 -> Prod4/4
  Constant4/1 -> Prod3/4
  Constant3/1 -> Prod2/3
  engine_speed_radps/1 -> Prod4/2, Prod4/1, Prod3/3, Prod2/2
  Prod4/1 -> Sum3/4
  Prod3/1 -> Sum3/3
  Prod2/1 -> Sum3/2
  Constant2/1 -> Sum3/1
  throttle_flow_gps/1 -> Sum1/1
  Sum1/1 -> Gain/1
  Gain/1 -> Prod1/1
  UnitDelay1/1 -> Prod4/3, Prod3/2, Prod3/1, Prod2/1, Sum2/2
  Sum2/1 -> UnitDelay1/1
  Prod1/1 -> Sum2/1
  Constant1/1 -> Prod1/2

== system fi_afc/Model 1/AF_Controller/fuel_controller/fuel_controller_10ms/feedback_PI_controller ==
  note: Feedback PI Controller
  airbyfuel_reference : Inport
  airbyfuel_meas : Inport  Port=2
  Enable : EnablePort
  Constant1 : Constant  Value=0.01  OutDataTypeStr=single  SampleTime=-1
      settings: AttributesFormatString=Sample Time [s]
  Gain : Gain  Gain=0.04  ParamDataTypeStr=single  OutDataTypeStr=Inherit: Inherit via back propagation  RndMeth=Simplest  SaturateOnIntegerOverflow=on
      settings: AttributesFormatString=Proportional Gain
  Gain1 : Gain  Gain=0.14  ParamDataTypeStr=single  OutDataTypeStr=Inherit: Inherit via back propagation  RndMeth=Simplest  SaturateOnIntegerOverflow=on
      settings: AttributesFormatString=Integral Gain
  Prod1 : Product  OutDataTypeStr=Inherit: Inherit via back propagation  RndMeth=Simplest
  Sum1 : Sum  Inputs=-+  OutDataTypeStr=Inherit: Inherit via back propagation  InputSameDT=on  RndMeth=Simplest
  Sum2 : Sum  OutDataTypeStr=Inherit: Inherit via back propagation  InputSameDT=on  RndMeth=Simplest
  Sum3 : Sum  OutDataTypeStr=Inherit: Inherit via back propagation  InputSameDT=on  RndMeth=Simplest
  UnitDelay1 : UnitDelay  SampleTime=-1
      settings: AttributesFormatString=Initial Value = 0
  closed_loop_fuel_trim : Outport  VectorParamsAs1DForOutWhenUnconnected=off
  wires:
  Gain/1 -> Sum3/1
  Sum3/1 -> closed_loop_fuel_trim/1
  Sum1/1 -> Gain1/1, Gain/1
  Gain1/1 -> Prod1/1
  Sum2/1 -> UnitDelay1/1, Sum3/2
  Constant1/1 -> Prod1/2
  airbyfuel_reference/1 -> Sum1/1
  airbyfuel_meas/1 -> Sum1/2
  Prod1/1 -> Sum2/1
  UnitDelay1/1 -> Sum2/2

== system fi_afc/Model 1/AF_Controller/fuel_controller/fuel_controller_10ms/feedforward_controller ==
  note: Feedforward Controller
  estimated_cyl_air_flow_gps : Inport
  airbyfuel_reference : Inport  Port=2
  Product : Product  Inputs=*/  RndMeth=Simplest  SaturateOnIntegerOverflow=on  OutDataTypeStr=Inherit: Same as first input
  desired_fuel_mass_gps : Outport  VectorParamsAs1DForOutWhenUnconnected=off
  wires:
  airbyfuel_reference/1 -> Product/2
  Product/1 -> desired_fuel_mass_gps/1
  estimated_cyl_air_flow_gps/1 -> Product/1

== system fi_afc/Model 1/AF_Controller/fuel_controller/fuel_controller_mode_10ms/normal_mode_detection ==
  note: Normal Mode Detection (Cold Start to Normal)
  note: NOTE: For first 10 seconds, controller uses only feedforward control to ignore the initialization issue.
  Logical Operator : Logic  Operator=OR  OutDataTypeStr=boolean
  Relational Operator : RelationalOperator  OutDataTypeStr=boolean  InputSameDT=off
  Sum : Sum
  Unit Delay1 : UnitDelay  SampleTime=-1
      settings: AttributesFormatString=Initial Value = 0
  Unit Delay2 : UnitDelay  SampleTime=-1
      settings: AttributesFormatString=Initial Value = 0
  normal_mode_start_sec : Constant  Value=10  OutDataTypeStr=single  SampleTime=-1
      settings: AttributesFormatString=Normal Mode Start Time (s)
  sampling_sec : Constant  Value=0.01  OutDataTypeStr=single  SampleTime=-1
      settings: AttributesFormatString=Sample Time (s)
  normal_on : Outport  VectorParamsAs1DForOutWhenUnconnected=off
  wires:
  Relational Operator/1 -> Logical Operator/1
  normal_mode_start_sec/1 -> Relational Operator/2
  Unit Delay1/1 -> Logical Operator/2
  Logical Operator/1 -> Unit Delay1/1, normal_on/1
  sampling_sec/1 -> Sum/2
  Unit Delay2/1 -> Sum/1
  Sum/1 -> Relational Operator/1, Unit Delay2/1

== system fi_afc/Model 1/AF_Controller/fuel_controller/fuel_controller_mode_10ms/power_mode_detection ==
  note: Power Mode Detection
  throttle_angle : Inport
  Constant : Constant  Value=50  OutDataTypeStr=single
      settings: AttributesFormatString=Base
  Constant1 : Constant  Value=20  OutDataTypeStr=single
      settings: AttributesFormatString=Hysteresis
  Relational Operator1 : RelationalOperator  OutDataTypeStr=boolean  InputSameDT=off
  Sum : Sum
  Switch : Switch  Criteria=u2 ~= 0  SaturateOnIntegerOverflow=off  InputSameDT=off
  Unit Delay1 : UnitDelay  SampleTime=-1
      settings: AttributesFormatString=Initial Value = 0
  power_on : Outport  VectorParamsAs1DForOutWhenUnconnected=off
  wires:
  Sum/1 -> Switch/3
  Constant1/1 -> Sum/2
  Constant/1 -> Switch/1, Sum/1
  throttle_angle/1 -> Relational Operator1/1
  Switch/1 -> Relational Operator1/2
  Unit Delay1/1 -> Switch/2
  Relational Operator1/1 -> power_on/1, Unit Delay1/1

== system fi_afc/Model 1/AF_Controller/fuel_controller/fuel_controller_mode_10ms/sensor_failure_detection ==
  note: A/F Sensor Failuer Detection
  airbyfuel_meas : Inport
  Logical Operator : Logic  Operator=OR  OutDataTypeStr=boolean
  Relational Operator : RelationalOperator  Operator=<=  OutDataTypeStr=boolean  InputSameDT=off
  Unit Delay : UnitDelay  SampleTime=-1
      settings: AttributesFormatString=Initial Value = 0
  threshold : Constant  Value=-1  OutDataTypeStr=single
  fail_on : Outport  VectorParamsAs1DForOutWhenUnconnected=off
  wires:
  Relational Operator/1 -> Logical Operator/1
  threshold/1 -> Relational Operator/2
  Unit Delay/1 -> Logical Operator/2
  Logical Operator/1 -> Unit Delay/1, fail_on/1
  airbyfuel_meas/1 -> Relational Operator/1
